simulink model "Boost_LQR_SIL"  (R2026a)
settings: Solver=FixedStepDiscrete  StopTime=0.05  FixedStep=Ts
InitFcn:
  | init_BOOT
values from neighbouring files (symbols this model uses):
  Ts = 250e-6    (= 0.00025)    [init_BOOT.m]
undefined symbols (not defined in the file or in its folder): den_Gp_d, dspblkCoreblockFVToolHelper, gcbh, num_Gp_d
settings Model: Creator=Usuario  LastModifiedBy=Usuario

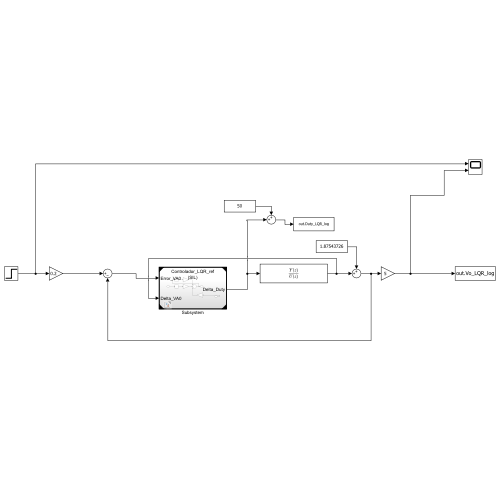
[thumbnail: Simulink's stored preview of the top-level diagram]
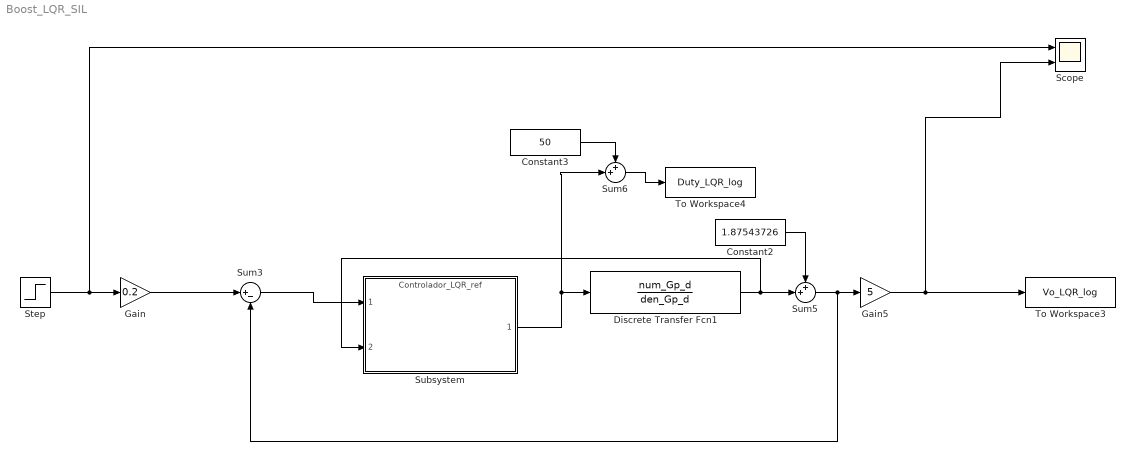
== system Boost_LQR_SIL ==
  Constant2 : Constant  Value=1.87543726
  Constant3 : Constant  Value=50
  Discrete Transfer Fcn1 : DiscreteTransferFcn  LoadFcn=dspblkCoreblockFVToolHelper(gcbh,'load');  Numerator=num_Gp_d  Denominator=den_Gp_d
      settings: CopyFcn=dspblkCoreblockFVToolHelper(gcbh,'copy');  DeleteFcn=dspblkCoreblockFVToolHelper(gcbh,'close');  ModelCloseFcn=dspblkCoreblockFVToolHelper(gcbh,'close');  PreSaveFcn=dspblkCoreblockFVToolHelper(gcbh,'presave');  PostSaveFcn=dspblkCoreblockFVToolHelper(gcbh,'postsave');  CloseFcn=dspblkCoreblockFVToolHelper(gcbh,'close');
  Gain : Gain  Gain=0.2
  Gain5 : Gain  Gain=5
  Scope : Scope  NumInputPorts=2
      settings: ActiveDisplayYMinimum=9.04733262947689  ActiveDisplayYMaximum=12.345869334708013
  Step : Step  Time=0.025  InitialValue=10  FinalValue=12  SampleTime=Ts
  Subsystem : ModelReference  ModelNameDialog=Controlador_LQR_ref  SimulationMode=Software-in-the-loop (SIL)  ModelReferenceVersion=1.6
  Sum3 : Sum  Inputs=|+-
  Sum5 : Sum  Inputs=++|
  Sum6 : Sum  Inputs=++|
  To Workspace3 : ToWorkspace  VariableName=Vo_LQR_log  SaveFormat=Timeseries  SampleTime=Ts
  To Workspace4 : ToWorkspace  VariableName=Duty_LQR_log  SaveFormat=Timeseries  SampleTime=Ts
  wires:
  Gain/1 -> Sum3/1
  Discrete Transfer Fcn1/1 -> Subsystem/2, Sum5/2
  Constant2/1 -> Sum5/1
  Sum5/1 -> Sum3/2, Gain5/1
  Constant3/1 -> Sum6/1
  Sum6/1 -> To Workspace4/1
  Step/1 -> Scope/1, Gain/1
  Gain5/1 -> Scope/2, To Workspace3/1
  Subsystem/1 -> Sum6/2, Discrete Transfer Fcn1/1
  Sum3/1 -> Subsystem/1
